simulink model "VLAClosedLoopControl"  (R2026a)
settings: Solver=VariableStepAuto  StopTime=40  FixedStep=1  MaxStep=0.02
undefined symbols (not defined in the file or in its folder): scenario
settings Model: Creator=smaddina  LastModifiedBy=smaddina

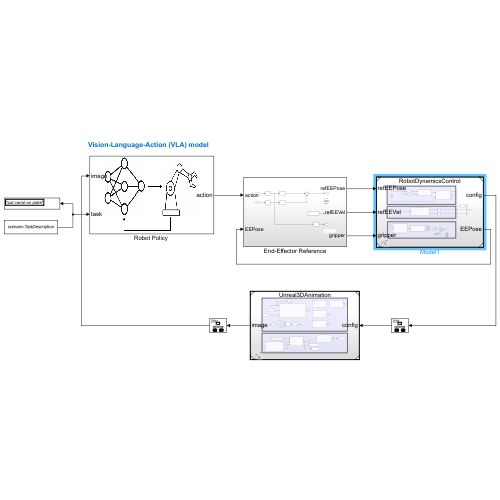
[thumbnail: Simulink's stored preview of the top-level diagram]
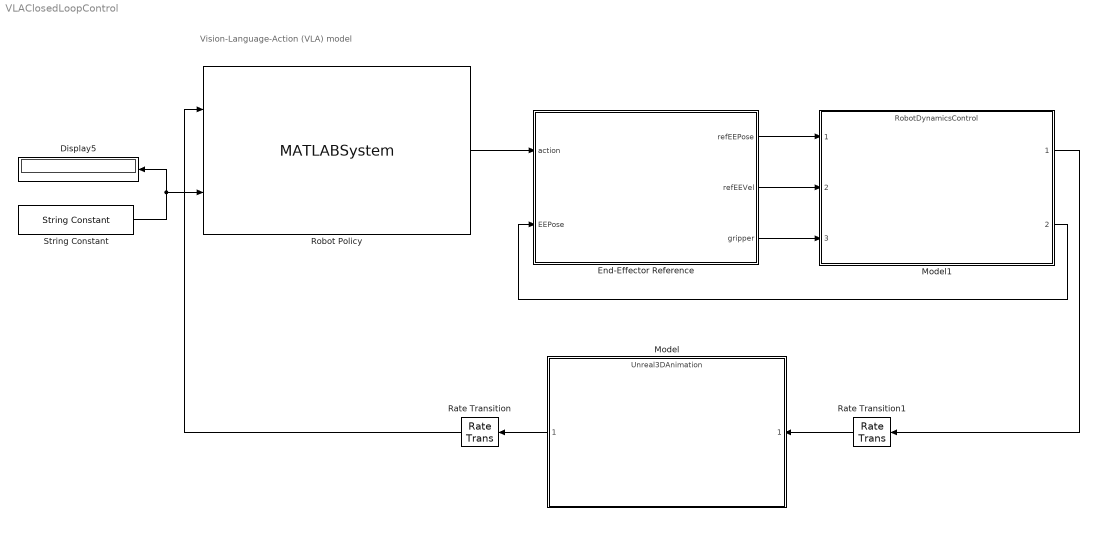
== system VLAClosedLoopControl ==
  note: Vision-Language-Action (VLA) model
  Display5 : Display
  End-Effector Reference : Subsystem
  Model : ModelReference  ModelNameDialog=Unreal3DAnimation.slx  SimulationMode=Normal  ModelReferenceVersion=4.13
  Model1 : ModelReference  ModelNameDialog=RobotDynamicsControl.slx  SimulationMode=Normal  ScheduleRatesWith=Schedule Editor  ModelReferenceVersion=4.22  CommunicationStepSize=0.02
  Rate Transition : RateTransition  InitialCondition=zeros(scenario.ImageSize(1),scenario.ImageSize(2),3,'uint8')  OutPortSampleTime=scenario.Ts
  Rate Transition1 : RateTransition  InitialCondition=scenario.RobotInitConfig  OutPortSampleTime=0.02
  "Robot Policy " : MATLABSystem  System=robotpolicy  ModelName=Octo
      mask Type: robotpolicy
  String Constant : StringConstant  String=scenario.TaskDescription
  wires:
  Model1/1 -> Rate Transition1/1
  Model/1 -> Rate Transition/1
  String Constant/1 -> Display5/1, "Robot Policy "/2
  "Robot Policy "/1 -> End-Effector Reference/1(action)
  Rate Transition/1 -> "Robot Policy "/1
  Rate Transition1/1 -> Model/1
  End-Effector Reference/1(refEEPose) -> Model1/1
  Model1/2 -> End-Effector Reference/2(EEPose)
  End-Effector Reference/2(refEEVel) -> Model1/2
  End-Effector Reference/3(gripper) -> Model1/3

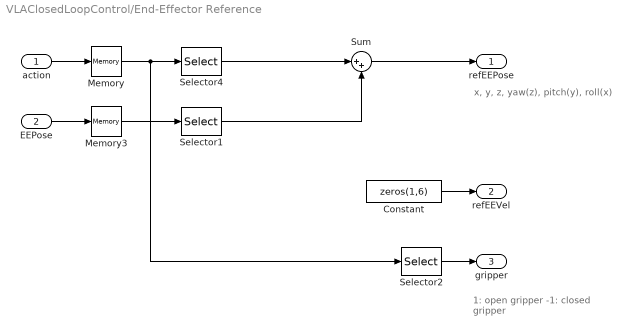
== system VLAClosedLoopControl/End-Effector Reference ==
  note: x, y, z,
      | yaw(z),
      | pitch(y),
      | roll(x)
  note: 1: open gripper
      | -1: closed gripper
  action : Inport
  EEPose : Inport  Port=2
  Constant : Constant  Value=zeros(1,6)
  Memory : Memory  InitialCondition=[zeros(scenario.NumStates-1,1); 1]  InheritSampleTime=on
  Memory3 : Memory  InitialCondition=scenario.RobotInitState  InheritSampleTime=on
  Selector1 : Selector  InputPortWidth=scenario.NumStates  IndexOptions=Index vector (dialog)  Indices=[1 2 3 4 5 6]  OutputSizes=1
  Selector2 : Selector  InputPortWidth=scenario.NumStates  IndexOptions=Index vector (dialog)  Indices=7  OutputSizes=1
  Selector4 : Selector  InputPortWidth=scenario.NumStates  IndexOptions=Index vector (dialog)  Indices=[1 2 3 4 5 6]  OutputSizes=1
  Sum : Sum  Inputs=|++
  refEEPose : Outport
  refEEVel : Outport  Port=2
  gripper : Outport  Port=3
  wires:
  Sum/1 -> refEEPose/1
  Selector2/1 -> gripper/1
  EEPose/1 -> Memory3/1
  Memory/1 -> Selector4/1, Selector2/1
  action/1 -> Memory/1
  Memory3/1 -> Selector1/1
  Selector4/1 -> Sum/1
  Selector1/1 -> Sum/2
  Constant/1 -> refEEVel/1
